simulink model "BatterySystemClosedLoop"  (R2026b)
settings: Solver=FixedStepDiscrete  StopTime=600  FixedStep=Ts
model workspace (MAT data in the model file):
  Ts = 1
  capacityAh = 1
  coolingCoefficient = 0.2
  initialSOC = 0.35
  initialTemperature = 25
  maxCurrent = 4
  reserveStop = 0.2
  resistance = 0.05
  thermalCapacity = 100
settings Model: Creator=mgado  LastModifiedBy=mgado

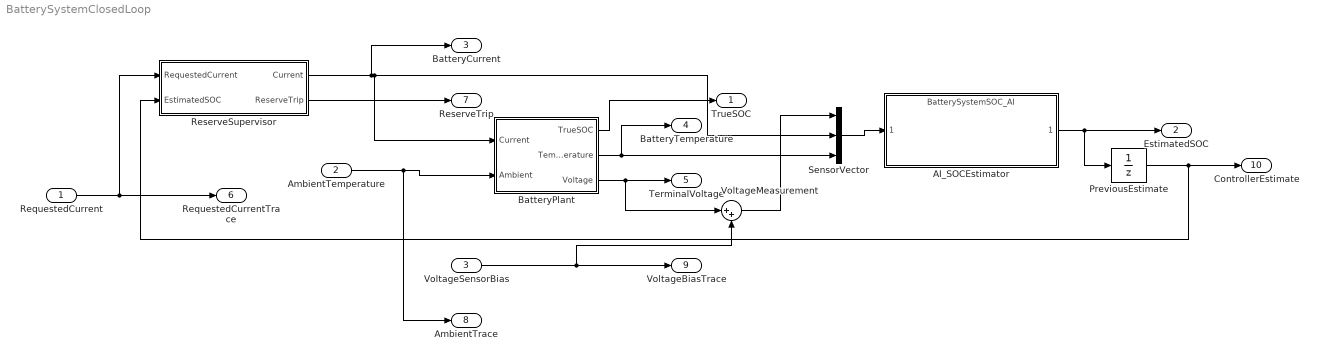
== system BatterySystemClosedLoop ==
  RequestedCurrent : Inport
  AmbientTemperature : Inport  Port=2
  VoltageSensorBias : Inport  Port=3
  AI_SOCEstimator : ModelReference  ModelNameDialog=BatterySystemSOC_AI  ModelReferenceVersion=1.1
  BatteryPlant : Subsystem
  PreviousEstimate : UnitDelay  InitialCondition=initialSOC  SampleTime=Ts
  ReserveSupervisor : Subsystem
  SensorVector : Mux  Inputs=3
  VoltageMeasurement : Sum  Inputs=|++
  TrueSOC : Outport
  EstimatedSOC : Outport  Port=2
  BatteryCurrent : Outport  Port=3
  BatteryTemperature : Outport  Port=4
  TerminalVoltage : Outport  Port=5
  RequestedCurrentTrace : Outport  Port=6
  ReserveTrip : Outport  Port=7
  AmbientTrace : Outport  Port=8
  VoltageBiasTrace : Outport  Port=9
  ControllerEstimate : Outport  Port=10
  wires:
  RequestedCurrent/1 -> RequestedCurrentTrace/1, ReserveSupervisor/1(RequestedCurrent)
  PreviousEstimate/1 -> ControllerEstimate/1, ReserveSupervisor/2(EstimatedSOC)
  ReserveSupervisor/1(Current) -> BatteryPlant/1(Current), SensorVector/2, BatteryCurrent/1
  AmbientTemperature/1 -> BatteryPlant/2(Ambient), AmbientTrace/1
  BatteryPlant/3(Voltage) -> TerminalVoltage/1, VoltageMeasurement/1
  VoltageSensorBias/1 -> VoltageBiasTrace/1, VoltageMeasurement/2
  VoltageMeasurement/1 -> SensorVector/1
  BatteryPlant/2(Temperature) -> BatteryTemperature/1, SensorVector/3
  SensorVector/1 -> AI_SOCEstimator/1
  AI_SOCEstimator/1 -> EstimatedSOC/1, PreviousEstimate/1
  BatteryPlant/1(TrueSOC) -> TrueSOC/1
  ReserveSupervisor/2(ReserveTrip) -> ReserveTrip/1

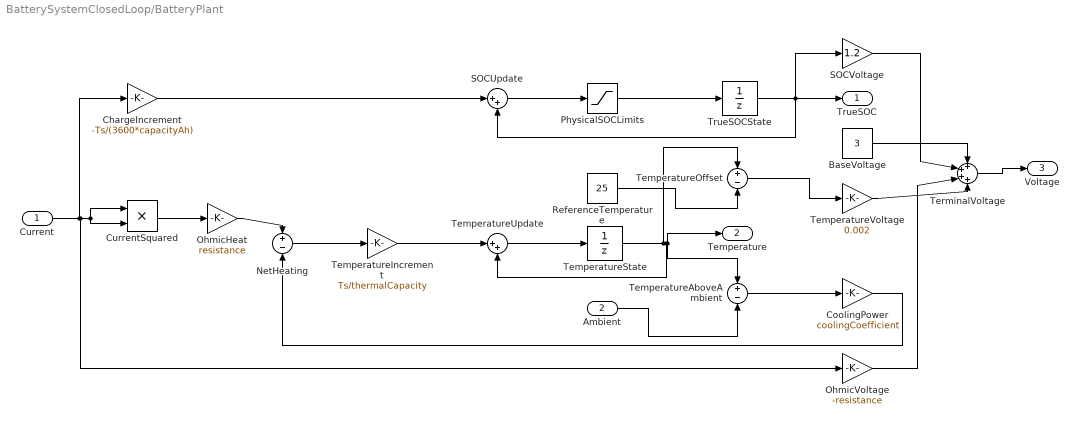
== system BatterySystemClosedLoop/BatteryPlant ==
  Current : Inport
  Ambient : Inport  Port=2
  BaseVoltage : Constant  Value=3
  ChargeIncrement : Gain  Gain=-Ts/(3600*capacityAh)
  CoolingPower : Gain  Gain=coolingCoefficient
  CurrentSquared : Product
  NetHeating : Sum  Inputs=+-
  OhmicHeat : Gain  Gain=resistance
  OhmicVoltage : Gain  Gain=-resistance
  PhysicalSOCLimits : Saturate  UpperLimit=1  LowerLimit=0
  ReferenceTemperature : Constant  Value=25
  SOCUpdate : Sum  Inputs=|++
  SOCVoltage : Gain  Gain=1.2
  TemperatureAboveAmbient : Sum  Inputs=+-
  TemperatureIncrement : Gain  Gain=Ts/thermalCapacity
  TemperatureOffset : Sum  Inputs=+-
  TemperatureState : UnitDelay  InitialCondition=initialTemperature  SampleTime=Ts
  TemperatureUpdate : Sum  Inputs=|++
  TemperatureVoltage : Gain  Gain=0.002
  TerminalVoltage : Sum  Inputs=++++
  TrueSOCState : UnitDelay  InitialCondition=initialSOC  SampleTime=Ts
  TrueSOC : Outport
  Temperature : Outport  Port=2
  Voltage : Outport  Port=3
  wires:
  TerminalVoltage/1 -> Voltage/1
  TemperatureVoltage/1 -> TerminalVoltage/4
  OhmicVoltage/1 -> TerminalVoltage/3
  SOCVoltage/1 -> TerminalVoltage/2
  BaseVoltage/1 -> TerminalVoltage/1
  TemperatureOffset/1 -> TemperatureVoltage/1
  ReferenceTemperature/1 -> TemperatureOffset/2
  TemperatureUpdate/1 -> TemperatureState/1
  TemperatureIncrement/1 -> TemperatureUpdate/1
  NetHeating/1 -> TemperatureIncrement/1
  CoolingPower/1 -> NetHeating/2
  OhmicHeat/1 -> NetHeating/1
  TemperatureAboveAmbient/1 -> CoolingPower/1
  Ambient/1 -> TemperatureAboveAmbient/2
  TemperatureState/1 -> Temperature/1, TemperatureAboveAmbient/1, TemperatureUpdate/2, TemperatureOffset/1
  CurrentSquared/1 -> OhmicHeat/1
  PhysicalSOCLimits/1 -> TrueSOCState/1
  SOCUpdate/1 -> PhysicalSOCLimits/1
  TrueSOCState/1 -> SOCUpdate/2, TrueSOC/1, SOCVoltage/1
  ChargeIncrement/1 -> SOCUpdate/1
  Current/1 -> CurrentSquared/1, CurrentSquared/2, OhmicVoltage/1, ChargeIncrement/1

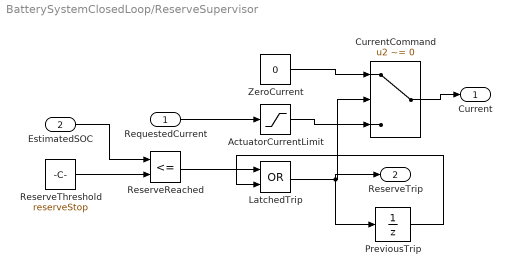
== system BatterySystemClosedLoop/ReserveSupervisor ==
  RequestedCurrent : Inport
  EstimatedSOC : Inport  Port=2
  ActuatorCurrentLimit : Saturate  UpperLimit=maxCurrent  LowerLimit=0
  CurrentCommand : Switch  Criteria=u2 ~= 0
  LatchedTrip : Logic  Operator=OR  IconShape=distinctive
  PreviousTrip : UnitDelay  SampleTime=Ts
  ReserveReached : RelationalOperator  Operator=<=
  ReserveThreshold : Constant  Value=reserveStop
  ZeroCurrent : Constant  Value=0
  Current : Outport
  ReserveTrip : Outport  Port=2
  wires:
  CurrentCommand/1 -> Current/1
  ActuatorCurrentLimit/1 -> CurrentCommand/3
  ZeroCurrent/1 -> CurrentCommand/1
  LatchedTrip/1 -> PreviousTrip/1, CurrentCommand/2, ReserveTrip/1
  PreviousTrip/1 -> LatchedTrip/2
  ReserveReached/1 -> LatchedTrip/1
  ReserveThreshold/1 -> ReserveReached/2
  EstimatedSOC/1 -> ReserveReached/1
  RequestedCurrent/1 -> ActuatorCurrentLimit/1
